simulink model "ellipsoidSMC"  (R2024a)
settings: Solver=ode45  StartTime=0  StopTime=350  FixedStep=0.01  MaxStep=0.01  RelTol=1e-4  AbsTol=1e-4  EnableMultiTasking=on
values from neighbouring files (symbols this model uses):
  simu = simulationClass()    [wecSimInputFile.m]
  waves = waveClass('regular')    [wecSimInputFile.m]
undefined symbols (not defined in the file or in its folder): body, controller, pto, X, Y, Z
libraries: nesl_utility x22, sm_lib x16, WECSim_Lib_Body_Elements x6, WECSim_Lib_Frames x1, vrlib x1, WECSim_Lib_PTOs x1
(part 3 of 3)

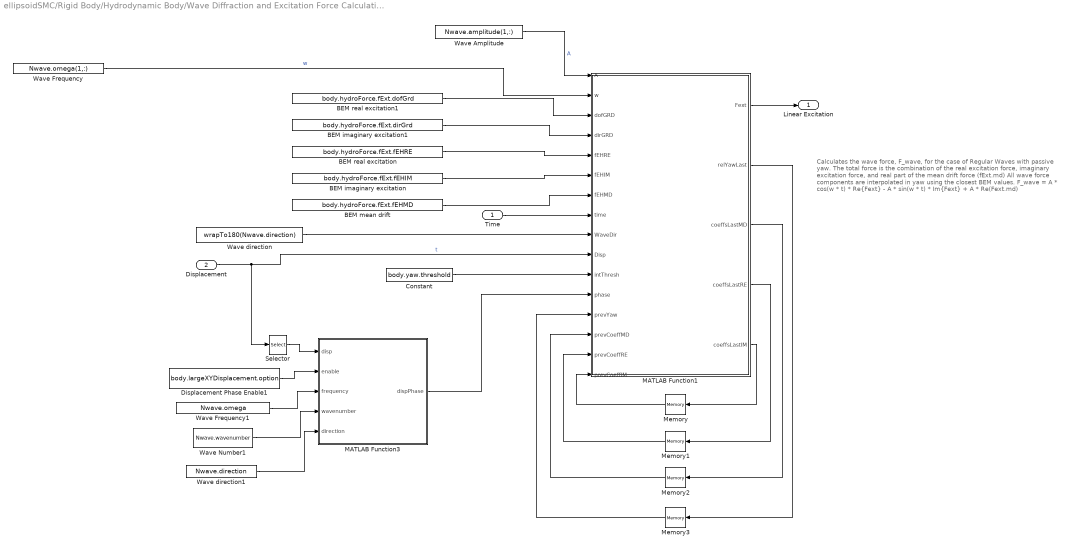
== system ellipsoidSMC/Rigid Body/Hydrodynamic Body/Wave Diffraction and Excitation Force Calculation/Linear Wave Excitation Force Variant Subsystem/Regular Wave NonLinear Yaw ==
  note: Calculates the wave force, F_wave, for the case of Regular Waves with passive yaw.
      |
      | The total force is the combination of the real excitation force, imaginary excitation force, and real part of the mean drift force (fExt.md)
      |
      | All wave force components are interpolated in yaw using the closest BEM values.
      |
      | F_wave =   A * cos(w * t) * Re{Fext}
      |                -  A * sin(w * t) * Im{Fext}
      |                + A * Re(Fext.md)
  Time : Inport
  Displacement : Inport  Port=2
  BEM imaginary excitation : Constant  Value=body.hydroForce.fExt.fEHIM  VectorParams1D=off
  BEM imaginary excitation1 : Constant  Value=body.hydroForce.fExt.dirGrd  VectorParams1D=off
  BEM mean drift : Constant  Value=body.hydroForce.fExt.fEHMD  VectorParams1D=off
  BEM real excitation : Constant  Value=body.hydroForce.fExt.fEHRE  VectorParams1D=off
  BEM real excitation1 : Constant  Value=body.hydroForce.fExt.dofGrd  VectorParams1D=off
  Constant : Constant  Value=body.yaw.threshold
  Displacement Phase Enable1 : Constant  Value=body.largeXYDisplacement.option
  MATLAB Function1 : MATLAB Function  TreatAsAtomicUnit=on
  MATLAB Function3 : MATLAB Function  TreatAsAtomicUnit=on
  Memory{,1..3} (4 alike) : Memory  InheritSampleTime=on  LinearizeAsDelay=on
  Selector : Selector  IndexOptions=Index vector (dialog)  Indices=[1 2]  OutputSizes=1
  Wave Amplitude : Constant  Value=Nwave.amplitude(1,:)
  Wave Frequency : Constant  Value=Nwave.omega(1,:)
  Wave Frequency1 : Constant  Value=Nwave.omega  VectorParams1D=off
  Wave Number1 : Constant  Value=Nwave.wavenumber
  Wave direction : Constant  Value=wrapTo180(Nwave.direction)  VectorParams1D=off
  Wave direction1 : Constant  Value=Nwave.direction  VectorParams1D=off
  Linear Excitation : Outport
  wires:
  Wave Frequency1/1 -> MATLAB Function3/3(frequency)
  Selector/1 -> MATLAB Function3/1(disp)
  Displacement Phase Enable1/1 -> MATLAB Function3/2(enable)
  Wave Number1/1 -> MATLAB Function3/4(wavenumber)
  Displacement/1 -> Selector/1, MATLAB Function1/10(Disp)  "t"
  Wave direction1/1 -> MATLAB Function3/5(direction)
  MATLAB Function3/1(dispPhase) -> MATLAB Function1/12(phase)
  Time/1 -> MATLAB Function1/8(time)
  MATLAB Function1/1(Fext) -> Linear Excitation/1
  Wave Frequency/1 -> MATLAB Function1/2(w)  "w"
  MATLAB Function1/5(coeffsLastIM) -> Memory/1
  MATLAB Function1/2(relYawLast) -> Memory3/1
  MATLAB Function1/4(coeffsLastRE) -> Memory1/1
  Memory3/1 -> MATLAB Function1/13(prevYaw)
  BEM mean drift/1 -> MATLAB Function1/7(fEHMD)
  Memory/1 -> MATLAB Function1/16(prevCoeffIM)
  Wave Amplitude/1 -> MATLAB Function1/1(A)  "A"
  MATLAB Function1/3(coeffsLastMD) -> Memory2/1
  BEM real excitation/1 -> MATLAB Function1/5(fEHRE)
  Wave direction/1 -> MATLAB Function1/9(WaveDir)
  BEM imaginary excitation/1 -> MATLAB Function1/6(fEHIM)
  BEM real excitation1/1 -> MATLAB Function1/3(dofGRD)
  Memory1/1 -> MATLAB Function1/15(prevCoeffRE)
  BEM imaginary excitation1/1 -> MATLAB Function1/4(dirGRD)
  Constant/1 -> MATLAB Function1/11(intThresh)
  Memory2/1 -> MATLAB Function1/14(prevCoeffMD)

== system ellipsoidSMC/Rigid Body/Hydrodynamic Body/Wave Diffraction and Excitation Force Calculation/Linear Wave Excitation Force Variant Subsystem/User Defined Wave Excitation Force ==
  note: Calculates the wave force, F_wave, for the case of User Defined Waves.
      |
      | F_wave = convolution calculation [1x6]
  InputWaveForceTimeHistory : FromWorkspace  VariableName=[Nwave.waveAmpTime(:,1),body.hydroForce.userDefinedFe]
  Linear Excitation : Outport
  wires:
  InputWaveForceTimeHistory/1 -> Linear Excitation/1

== system ellipsoidSMC/Rigid Body/Hydrodynamic Body/Wave Diffraction and Excitation Force Calculation/Nonlinear FK Force Variant Subsystem/No Nonlinear FroudeKrylov Force ==
  Constant : Constant  Value=zeros(1,body.dof)
  Nonlinear Excitation : Outport
  wires:
  Constant/1 -> Nonlinear Excitation/1

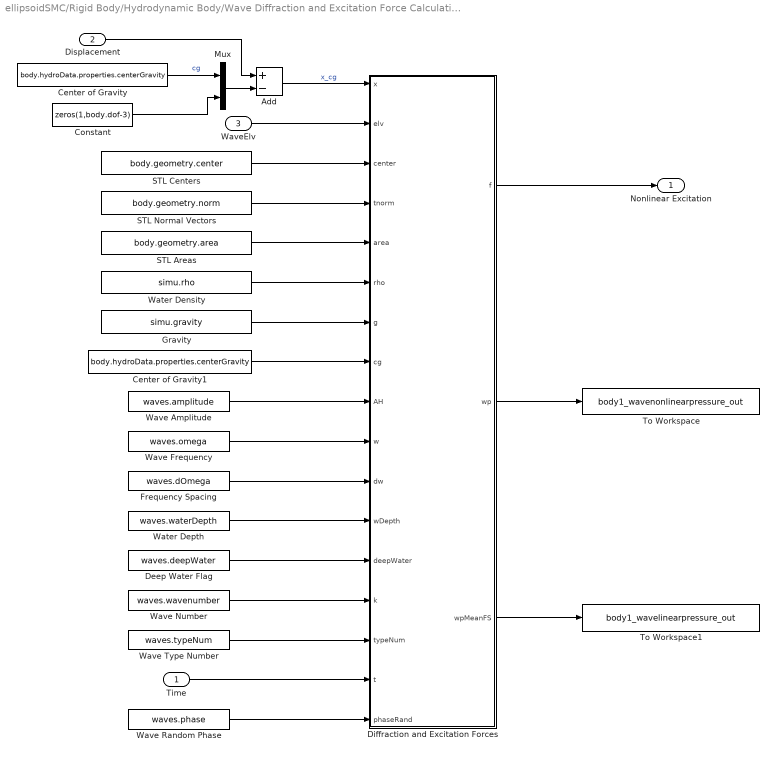
== system ellipsoidSMC/Rigid Body/Hydrodynamic Body/Wave Diffraction and Excitation Force Calculation/Nonlinear FK Force Variant Subsystem/With Nonlinear FroudeKrylov Force ==
  Time : Inport
  Displacement : Inport  Port=2
  WaveElv : Inport  Port=3
  Add : Sum  Inputs=+-
  Center of Gravity : Constant  Value=body.hydroData.properties.centerGravity
  Center of Gravity1 : Constant  Value=body.hydroData.properties.centerGravity
  Constant : Constant  Value=zeros(1,body.dof-3)
  Deep Water Flag : Constant  Value=waves.deepWater
  Diffraction and Excitation Forces : MATLAB Function  TreatAsAtomicUnit=on
  Frequency Spacing : Constant  Value=waves.dOmega
  Gravity : Constant  Value=simu.gravity
  Mux : Mux  Inputs=2
  STL Areas : Constant  Value=body.geometry.area
  STL Centers : Constant  Value=body.geometry.center
  STL Normal Vectors : Constant  Value=body.geometry.norm
  To Workspace : ToWorkspace  VariableName=body1_wavenonlinearpressure_out  SaveFormat=Structure With Time  SampleTime=-1
      settings: Decimation=round(simu.dtOut/simu.dt,0)
  To Workspace1 : ToWorkspace  VariableName=body1_wavelinearpressure_out  SaveFormat=Structure With Time  SampleTime=-1
      settings: Decimation=round(simu.dtOut/simu.dt,0)
  Water Density : Constant  Value=simu.rho
  Water Depth : Constant  Value=waves.waterDepth
  Wave Amplitude : Constant  Value=waves.amplitude
  Wave Frequency : Constant  Value=waves.omega
  Wave Number : Constant  Value=waves.wavenumber
  Wave Random Phase : Constant  Value=waves.phase
  Wave Type Number : Constant  Value=waves.typeNum
  Nonlinear Excitation : Outport
  wires:
  STL Areas/1 -> Diffraction and Excitation Forces/5(area)
  Diffraction and Excitation Forces/2(wp) -> To Workspace/1
  Diffraction and Excitation Forces/3(wpMeanFS) -> To Workspace1/1
  Displacement/1 -> Add/1
  Constant/1 -> Mux/2
  Center of Gravity/1 -> Mux/1  "cg"
  Mux/1 -> Add/2
  Add/1 -> Diffraction and Excitation Forces/1(x)  "x_cg"
  Deep Water Flag/1 -> Diffraction and Excitation Forces/13(deepWater)
  Wave Random Phase/1 -> Diffraction and Excitation Forces/17(phaseRand)
  Water Depth/1 -> Diffraction and Excitation Forces/12(wDepth)
  Wave Number/1 -> Diffraction and Excitation Forces/14(k)
  Wave Type Number/1 -> Diffraction and Excitation Forces/15(typeNum)
  Frequency Spacing/1 -> Diffraction and Excitation Forces/11(dw)
  Wave Frequency/1 -> Diffraction and Excitation Forces/10(w)
  Wave Amplitude/1 -> Diffraction and Excitation Forces/9(AH)
  Time/1 -> Diffraction and Excitation Forces/16(t)
  WaveElv/1 -> Diffraction and Excitation Forces/2(elv)
  STL Centers/1 -> Diffraction and Excitation Forces/3(center)
  STL Normal Vectors/1 -> Diffraction and Excitation Forces/4(tnorm)
  Water Density/1 -> Diffraction and Excitation Forces/6(rho)
  Gravity/1 -> Diffraction and Excitation Forces/7(g)
  Diffraction and Excitation Forces/1(f) -> Nonlinear Excitation/1
  Center of Gravity1/1 -> Diffraction and Excitation Forces/8(cg)

== system ellipsoidSMC/Rigid Body/Hydrodynamic Body/Wave Radiation Forces Calculation/SS CI and Constant-Damping-CoeVariant Subsystem/Constant Coefficients ==
  note: F = damping * velocity
  velocity : Inport
  Product : Product  Multiplication=Matrix(*)
  Radiation Damping Matrix : Constant  Value=body.hydroForce.fDamping
  Out1 : Outport
  wires:
  velocity/1 -> Product/2
  Product/1 -> Out1/1  "F_Single Frequency"
  Radiation Damping Matrix/1 -> Product/1

== system ellipsoidSMC/Rigid Body/Hydrodynamic Body/Wave Radiation Forces Calculation/SS CI and Constant-Damping-CoeVariant Subsystem/Convolution Integral Calculation ==
  note: Calculate the convolution integral using the radiation IRF (body.hydroForce.irkb) and the velocity.
  velocity : Inport
  IRBK : Constant  Value=body.hydroForce.irkb
  MATLAB Function1 : MATLAB Function  TreatAsAtomicUnit=on  SystemSampleTime=simu.cicTime(2)-simu.cicTime(1)
  Rate Transition : RateTransition
  Reshape : Reshape
  cicTime : Constant  Value=simu.cicTime
  Out1 : Outport
  wires:
  velocity/1 -> MATLAB Function1/1(velocity)
  cicTime/1 -> MATLAB Function1/3(cicTime)
  IRBK/1 -> MATLAB Function1/2(IRKB)
  MATLAB Function1/1(F_FM) -> Rate Transition/1
  Rate Transition/1 -> Reshape/1
  Reshape/1 -> Out1/1

== system ellipsoidSMC/Rigid Body/Hydrodynamic Body/Wave Radiation Forces Calculation/SS CI and Constant-Damping-CoeVariant Subsystem/FIR Filter Calculation ==
  velocity : Inport
  FIR Filter Matrix : Subsystem  mask{B2B=simu.b2b, body=body}
      mask prompts: body "bodyClass"
      mask init:
      | if exist('body','var')
      |     TotalRows = body.dof;
      |     
      |     cb = gcb;
      |     
      |     set_param([cb '/Mux'],...
      |                'Inputs',sprintf('%d',TotalRows));
      |     
      |     set_param([cb '/FIR_filter_row'],...
      |                'position',[0, 100, 200, 140]);
      |     
      |     set_param([cb '/FIR_filter_row'],...
      |                'rowNo', '1');
      |     
      |     try
      |     add_line(cb,...
      |             ['velocity','/1'], ...    
      |             'FIR_filter_row/1',... 
      |             'autorouting','on');
      |     catch
      |     end
      |     
      |     try
      |     add_line(cb,...
      |             ['FIR_filter_row','/1'], ...    
      |             'Mux/1',... 
      |             'autorouting','on');
      |     catch
      |     end
      |     
      |     for i = 2:TotalRows
      |         add_block([cb,'/FIR_filter_row'],[cb,'/FIR_filter_row',num2str(i)], 'MakeNameUnique','off');
      |         set_param([cb '/FIR_filter_row',num2str(i)],...
      |                    'position',[0, 100*i, 200, 40 + 100*i]);
      |         set_param([cb '/FIR_filter_row',num2str(i)],...
      |                    'rowNo', num2str(i));
      |         add_line(cb,...
      |                 ['velocity','/1'], ...    
      |                 ['FIR_filter_row',num2str(i),'/1'],... 
      |                 'autorouting','on');
      |         add_line(cb,...
      |                 ['FIR_filter_row',num2str(i),'/1'], ...    
      |                 ['Mux/',num2str(i)],... 
      |                 'autorouting','on');
      |     end
      | end
  Rate Transition : RateTransition  OutPortSampleTime=simu.cicDt
  Rate Transition1 : RateTransition  OutPortSampleTime=simu.cicDt
  Out1 : Outport
  wires:
  Rate Transition1/1 -> Out1/1
  Rate Transition/1 -> FIR Filter Matrix/1(velocity)
  FIR Filter Matrix/1(Out1) -> Rate Transition1/1
  velocity/1 -> Rate Transition/1

== system ellipsoidSMC/Rigid Body/Hydrodynamic Body/Wave Radiation Forces Calculation/SS CI and Constant-Damping-CoeVariant Subsystem/State-Space Calculation  ==
  note: Calculate the radiation damping based on the state space formulation. Coefficients are defined in body.hydroForce.ssRadf
  velocity : Inport
  State-Space : StateSpace  A=body.hydroForce.ssRadf.A  B=body.hydroForce.ssRadf.B  C=body.hydroForce.ssRadf.C  D=body.hydroForce.ssRadf.D  InitialCondition=0
  Out1 : Outport
  wires:
  State-Space/1 -> Out1/1
  velocity/1 -> State-Space/1  "x"

== system ellipsoidSMC/Rigid Body/Hydrodynamic Body/Hydrostatic Restoring Force Calculation/Linear and Nonlinear Restoring Force Variant Subsystem/Linear Hydrostatic Restoring Force/Net Buoyancy Force ==
  note: The total buoyancy force is due to the vertical buoyancy force (gravity - buoyancy) and a rotational buoyancy force if the center of gravity is not aligned with the center of buoyancy.
      |
      | F_NetBuoyancy = F_gravity - F_buoyancy + F_rotational_buoyancy
      |
      | F_rotational_buoyancy = (cb-cg) x F_buoyancy
      | F_buoyancy = rho*g*V_0
      | F_gravity = m*g
  Body Mass : Inport
  Add1 : Sum  Inputs=+-
  Add2 : Sum
  Add3 : Sum  Inputs=+-
  Assignment (Add Net Bouyancy Force to Z-Direction) : Assignment  IndexOptions=Index vector (dialog)  Indices=3  OutputSizes=1
  Assignment (Add Net Bouyancy Force to Z-Direction)1 : Assignment  IndexOptions=Index vector (dialog)  Indices=3  OutputSizes=1
  Assignment (Add Net Bouyancy Force to Z-Direction)2 : Assignment  IndexOptions=Index vector (dialog)  Indices=4:6  OutputSizes=1
  Center of Buoyancy : Constant  Value=body.centerBuoyancy
  Center of Gravity : Constant  Value=body.centerGravity
  Constant1 : Constant  Value=zeros(1,body.dof)
  Constant2 : Constant  Value=[0 0 0]
  Cross Product : vrlib/Utilities/Cross Product
  Gravity : Constant  Value=simu.gravity
  Product : Product
  Product1 : Product  Inputs=3
  Volume : Constant  Value=body.volume
  Water Density : Constant  Value=simu.rho
  F_NetBuoyancy : Outport
  wires:
  Add1/1 -> Assignment (Add Net Bouyancy Force to Z-Direction)/2
  Body Mass/1 -> Product/2  "m"
  Cross Product/1 -> Assignment (Add Net Bouyancy Force to Z-Direction)2/2
  Add2/1 -> F_NetBuoyancy/1  "Net buoyancy force"
  Add3/1 -> Cross Product/2
  Constant2/1 -> Assignment (Add Net Bouyancy Force to Z-Direction)1/1
  Center of Gravity/1 -> Add3/2  "cg"
  Constant1/1 -> Assignment (Add Net Bouyancy Force to Z-Direction)/1, Assignment (Add Net Bouyancy Force to Z-Direction)2/1
  Center of Buoyancy/1 -> Add3/1  "x"
  Assignment (Add Net Bouyancy Force to Z-Direction)1/1 -> Cross Product/1
  Volume/1 -> Product1/3  "Vol"
  Assignment (Add Net Bouyancy Force to Z-Direction)/1 -> Add2/1  "Vertical Buoyancy Force"
  Water Density/1 -> Product1/1  "rho"
  Gravity/1 -> Product/1, Product1/2  "g"
  Product1/1 -> Assignment (Add Net Bouyancy Force to Z-Direction)1/2, Add1/2  "F_Buoyancy"
  Product/1 -> Add1/1  "F_Gravity"
  Assignment (Add Net Bouyancy Force to Z-Direction)2/1 -> Add2/2  "Rotational buoyancy force"

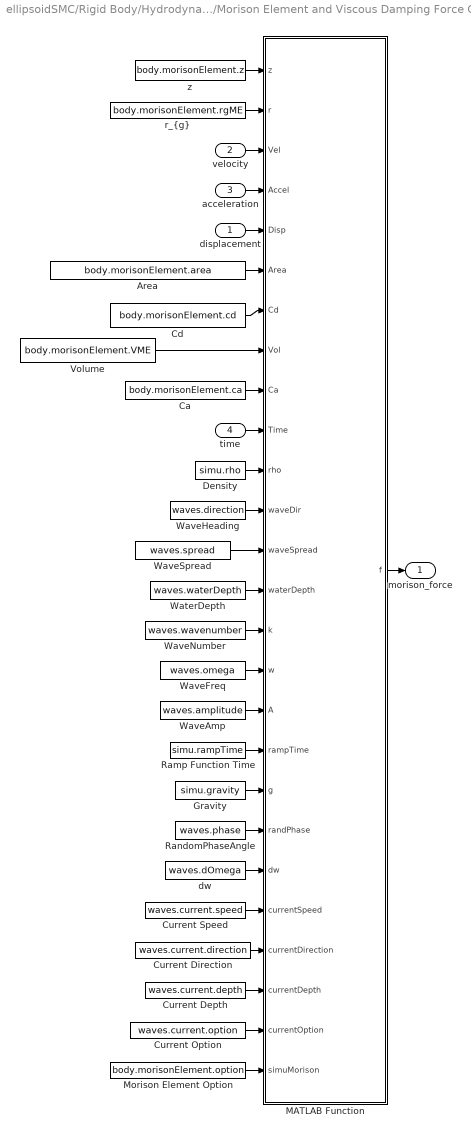
== system ellipsoidSMC/Rigid Body/Hydrodynamic Body/Morison Element and Viscous Damping Force Calculation/Morison Element Variant Subsystem/Morison Element On/Irregular Wave Morison Force ==
  displacement : Inport
  velocity : Inport  Port=2
  acceleration : Inport  Port=3
  time : Inport  Port=4
  Area : Constant  Value=body.morisonElement.area  VectorParams1D=off
  Ca : Constant  Value=body.morisonElement.ca  VectorParams1D=off
  Cd : Constant  Value=body.morisonElement.cd  VectorParams1D=off
  Current Depth : Constant  Value=waves.current.depth
  Current Direction : Constant  Value=waves.current.direction
  Current Option : Constant  Value=waves.current.option
  Current Speed : Constant  Value=waves.current.speed
  Density : Constant  Value=simu.rho
  Gravity : Constant  Value=simu.gravity
  MATLAB Function : MATLAB Function  TreatAsAtomicUnit=on
  Morison Element Option : Constant  Value=body.morisonElement.option
  Ramp Function Time : Constant  Value=simu.rampTime
  RandomPhaseAngle : Constant  Value=waves.phase  VectorParams1D=off
  Volume : Constant  Value=body.morisonElement.VME  VectorParams1D=off
  WaterDepth : Constant  Value=waves.waterDepth
  WaveAmp : Constant  Value=waves.amplitude
  WaveFreq : Constant  Value=waves.omega
  WaveHeading : Constant  Value=waves.direction
  WaveNumber : Constant  Value=waves.wavenumber
  WaveSpread : Constant  Value=waves.spread
  dw : Constant  Value=waves.dOmega  VectorParams1D=off
  "r_{g}" : Constant  Value=body.morisonElement.rgME  VectorParams1D=off
  z : Constant  Value=body.morisonElement.z  VectorParams1D=off
  morison_force : Outport
  wires:
  WaveSpread/1 -> MATLAB Function/13(waveSpread)
  Morison Element Option/1 -> MATLAB Function/26(simuMorison)
  Current Option/1 -> MATLAB Function/25(currentOption)
  Current Depth/1 -> MATLAB Function/24(currentDepth)
  Current Direction/1 -> MATLAB Function/23(currentDirection)
  Current Speed/1 -> MATLAB Function/22(currentSpeed)
  dw/1 -> MATLAB Function/21(dw)
  RandomPhaseAngle/1 -> MATLAB Function/20(randPhase)
  Gravity/1 -> MATLAB Function/19(g)
  Ramp Function Time/1 -> MATLAB Function/18(rampTime)
  WaveAmp/1 -> MATLAB Function/17(A)
  WaveFreq/1 -> MATLAB Function/16(w)
  WaveNumber/1 -> MATLAB Function/15(k)
  WaterDepth/1 -> MATLAB Function/14(waterDepth)
  WaveHeading/1 -> MATLAB Function/12(waveDir)
  Density/1 -> MATLAB Function/11(rho)
  time/1 -> MATLAB Function/10(Time)
  Ca/1 -> MATLAB Function/9(Ca)
  Volume/1 -> MATLAB Function/8(Vol)
  Cd/1 -> MATLAB Function/7(Cd)
  Area/1 -> MATLAB Function/6(Area)
  displacement/1 -> MATLAB Function/5(Disp)
  acceleration/1 -> MATLAB Function/4(Accel)
  velocity/1 -> MATLAB Function/3(Vel)
  "r_{g}"/1 -> MATLAB Function/2(r)
  z/1 -> MATLAB Function/1(z)
  MATLAB Function/1(f) -> morison_force/1

== system ellipsoidSMC/Rigid Body/Hydrodynamic Body/Morison Element and Viscous Damping Force Calculation/Morison Element Variant Subsystem/Morison Element On/No Wave Morison Force ==
  displacement : Inport
  velocity : Inport  Port=2
  acceleration : Inport  Port=3
  time : Inport  Port=4
  Area : Constant  Value=body.morisonElement.area  VectorParams1D=off
  Ca : Constant  Value=body.morisonElement.ca  VectorParams1D=off
  Cd : Constant  Value=body.morisonElement.cd  VectorParams1D=off
  Current Depth : Constant  Value=waves.current.depth
  Current Direction : Constant  Value=waves.current.direction
  Current Option : Constant  Value=waves.current.option
  Current Speed : Constant  Value=waves.current.speed
  Density : Constant  Value=simu.rho
  Morison Element Option : Constant  Value=body.morisonElement.option
  MorisonElement(s) : MATLAB Function  TreatAsAtomicUnit=on
  Ramp Function Time : Constant  Value=simu.rampTime
  Volume : Constant  Value=body.morisonElement.VME  VectorParams1D=off
  "r_{g}" : Constant  Value=body.morisonElement.rgME  VectorParams1D=off
  z : Constant  Value=body.morisonElement.z  VectorParams1D=off
  morison_force : Outport
  wires:
  Morison Element Option/1 -> MorisonElement(s)/17(bodyMorison)
  Current Option/1 -> MorisonElement(s)/16(currentOption)
  Current Depth/1 -> MorisonElement(s)/15(currentDepth)
  Current Direction/1 -> MorisonElement(s)/14(currentDirection)
  Current Speed/1 -> MorisonElement(s)/13(currentSpeed)
  Ramp Function Time/1 -> MorisonElement(s)/12(rampTime)
  Density/1 -> MorisonElement(s)/11(rho)
  time/1 -> MorisonElement(s)/10(Time)
  Ca/1 -> MorisonElement(s)/9(Ca)
  Volume/1 -> MorisonElement(s)/8(Vol)
  Cd/1 -> MorisonElement(s)/7(Cd)
  Area/1 -> MorisonElement(s)/6(Area)
  displacement/1 -> MorisonElement(s)/5(Disp)
  acceleration/1 -> MorisonElement(s)/4(Accel)
  velocity/1 -> MorisonElement(s)/3(Vel)
  "r_{g}"/1 -> MorisonElement(s)/2(r)
  z/1 -> MorisonElement(s)/1(z)
  MorisonElement(s)/1(f) -> morison_force/1

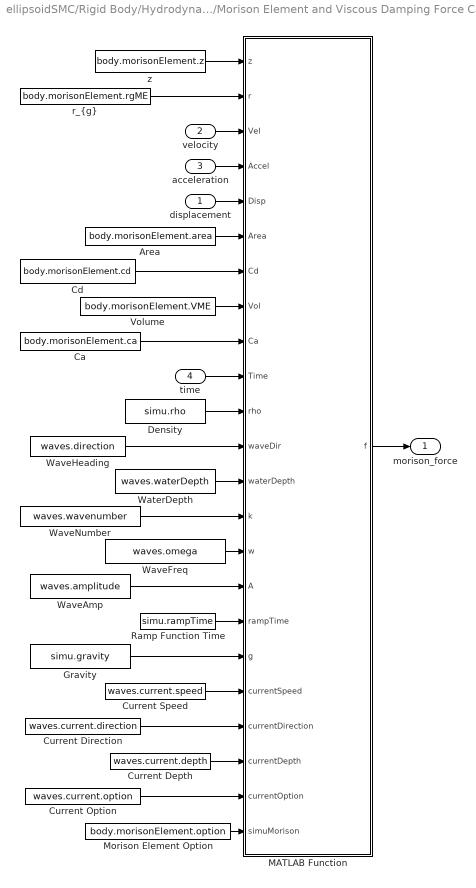
== system ellipsoidSMC/Rigid Body/Hydrodynamic Body/Morison Element and Viscous Damping Force Calculation/Morison Element Variant Subsystem/Morison Element On/Regular Wave Morison Force ==
  displacement : Inport
  velocity : Inport  Port=2
  acceleration : Inport  Port=3
  time : Inport  Port=4
  Area : Constant  Value=body.morisonElement.area  VectorParams1D=off
  Ca : Constant  Value=body.morisonElement.ca  VectorParams1D=off
  Cd : Constant  Value=body.morisonElement.cd  VectorParams1D=off
  Current Depth : Constant  Value=waves.current.depth
  Current Direction : Constant  Value=waves.current.direction
  Current Option : Constant  Value=waves.current.option
  Current Speed : Constant  Value=waves.current.speed
  Density : Constant  Value=simu.rho
  Gravity : Constant  Value=simu.gravity
  MATLAB Function : MATLAB Function  TreatAsAtomicUnit=on
  Morison Element Option : Constant  Value=body.morisonElement.option
  Ramp Function Time : Constant  Value=simu.rampTime
  Volume : Constant  Value=body.morisonElement.VME  VectorParams1D=off
  WaterDepth : Constant  Value=waves.waterDepth
  WaveAmp : Constant  Value=waves.amplitude
  WaveFreq : Constant  Value=waves.omega
  WaveHeading : Constant  Value=waves.direction
  WaveNumber : Constant  Value=waves.wavenumber
  "r_{g}" : Constant  Value=body.morisonElement.rgME  VectorParams1D=off
  z : Constant  Value=body.morisonElement.z  VectorParams1D=off
  morison_force : Outport
  wires:
  Current Speed/1 -> MATLAB Function/19(currentSpeed)
  WaveAmp/1 -> MATLAB Function/16(A)
  Gravity/1 -> MATLAB Function/18(g)
  WaveNumber/1 -> MATLAB Function/14(k)
  Ca/1 -> MATLAB Function/9(Ca)
  Current Direction/1 -> MATLAB Function/20(currentDirection)
  Area/1 -> MATLAB Function/6(Area)
  WaterDepth/1 -> MATLAB Function/13(waterDepth)
  acceleration/1 -> MATLAB Function/4(Accel)
  Density/1 -> MATLAB Function/11(rho)
  WaveHeading/1 -> MATLAB Function/12(waveDir)
  WaveFreq/1 -> MATLAB Function/15(w)
  Cd/1 -> MATLAB Function/7(Cd)
  displacement/1 -> MATLAB Function/5(Disp)
  Current Option/1 -> MATLAB Function/22(currentOption)
  Current Depth/1 -> MATLAB Function/21(currentDepth)
  time/1 -> MATLAB Function/10(Time)
  "r_{g}"/1 -> MATLAB Function/2(r)
  Ramp Function Time/1 -> MATLAB Function/17(rampTime)
  velocity/1 -> MATLAB Function/3(Vel)
  Volume/1 -> MATLAB Function/8(Vol)
  Morison Element Option/1 -> MATLAB Function/23(simuMorison)
  z/1 -> MATLAB Function/1(z)
  MATLAB Function/1(f) -> morison_force/1

== system ellipsoidSMC/Rigid Body/Hydrodynamic Body/Wave Radiation Forces Calculation/SS CI and Constant-Damping-CoeVariant Subsystem/FIR Filter Calculation/FIR Filter Matrix ==
  velocity : Inport
  FIR_filter_row : Subsystem  mask{body=body, B2B=simu.b2b, rowNo=1}
      mask prompts: body "BodyClass"
      mask init:
      | cb = gcb;
      | % The implementation that follows, calculates the radiation force, Fr, by
      | % calculating the Fr for each body mode by multiplying the velocity vector
      | % to the IRF matrix -- whose each row corresponds to the Fr for each of the
      | % modes corresponding to the velocity vector.
      | 
      | 
      | % Get the radiation IRF coefficients using body.hydroForce.irkb
      | set_param([cb '/Discrete FIR Filter'],...
      |            'position',[100, 0, 140, 180]);
      |          if rem(rowNo,6) ~= 0
      |         set_param([cb,'/Discrete FIR Filter'],...
      |                   'Coefficients', [sprintf('transpose(squeeze(body.hydroForce.irkb(:,%d,%d)))',rem(rowNo,6),1)]); 
      |          elseif rem(rowNo,6) == 0
      |         set_param([cb,'/Discrete FIR Filter'],...
      |                   'Coefficients', [sprintf('transpose(squeeze(body.hydroForce.irkb(:,%d,%d)))',6,1)]); 
      |          end
      | % Assign number of filters. The number of filter corresponds to the IRF
      | % matrix elements being used for the calculation for each row.
      | nFilt = body.dof + B2B*(body.total-1)*6;
      | 
      | % Add Demux channels corresponding to number of filters, and connect them to the corresponding filter.
      | 
      | set_param([cb '/Demux'],...
      |            'Outputs',sprintf('%d',nFilt));
      | try
      | add_line(cb,...
      |         'Demux/1',...
      |         ['Discrete FIR Filter','/1'], ...     
      |         'autorouting','on');
      | catch
      | end
      | 
      | try
      | add_line(cb,...
      |         'Discrete FIR Filter/1', ...     
      |         'Add/1',...
      |         'autorouting','on');
      | catch 
      | end
      | 
      | % Add filters 
      | 
      | for i = 2:nFilt
      | 
      |      try
      |         add_block([cb,'/Discrete FIR Filter'],[cb,'/Discrete FIR Filter ',num2str(i)],'MakeNameUnique','off',...
      |                    'Position',[100*i, 0, 40+100*i, 180],'BackgroundColor','white');
      |         signlist = get_param([cb,'/Add'],'Inputs');
      |         set_param([cb,'/Add'],'Inputs',[signlist,'+']);
      |      catch 
      |      end
      | 
      | 
      |      try
      |          if rem(rowNo,6) ~= 0
      |         set_param([cb,'/Discrete FIR Filter ',num2str(i)],...
      |                   'Coefficients', [sprintf('transpose(squeeze(body.hydroForce.irkb(:,%d,%d)))',rem(rowNo,6),i)]); 
      |          elseif rem(rowNo,6) == 0
      |         set_param([cb,'/Discrete FIR Filter ',num2str(i)],...
      |                   'Coefficients', [sprintf('transpose(squeeze(body.hydroForce.irkb(:,%d,%d)))',6,i)]); 
      |          end
      |      catch
      |      end
      | 
      |      try
      |         add_line(cb,...
      |         ['Demux/',num2str(i)],...
      |         ['Discrete FIR Filter ',num2str(i),'/1'], ...     
      |         'autorouting','on');
      |      catch
      |      end
      | 
      | 
      |      try
      |         add_line(cb,...
      |         ['Discrete FIR Filter ',num2str(i),'/1'], ...     
      |         ['Add/', num2str(i)],...
      |         'autorouting','on');
      |     catch 
      |     end
      | end
  Gain : Gain  Gain=simu.cicDt
  Mux : Mux  Inputs=1
  Out1 : Outport
  wires:
  Gain/1 -> Out1/1
  FIR_filter_row/1(Out1) -> Mux/1
  velocity/1 -> FIR_filter_row/1(In1)
  Mux/1 -> Gain/1

== system ellipsoidSMC/Rigid Body/Hydrodynamic Body/Wave Radiation Forces Calculation/SS CI and Constant-Damping-CoeVariant Subsystem/FIR Filter Calculation/FIR Filter Matrix/FIR_filter_row ==
  In1 : Inport
  Add : Sum  Inputs=+
  Demux : Demux  Outputs=1
      settings: AttributesFormatString=%<Outputs>
  Discrete FIR Filter : DiscreteFir  Coefficients=transpose(squeeze(body.hydroForce.irkb(:,1,1)))
  Out1 : Outport
  wires:
  Add/1 -> Out1/1
  In1/1 -> Demux/1

== matlab function ellipsoidSMC/Rigid Body/Hydrodynamic Body/Morison Element and Viscous Damping Force Calculation/Morison Element Variant Subsystem/Morison Element On/No Wave Morison Force/MorisonElement(s) ==
  data: z input; f output; r input; Vel input; Accel input; Disp input; Area input; Cd input; Vol input; Ca input; Time input; rho input; rampTime input; currentSpeed input; currentDirection input; currentDepth input; currentOption input; bodyMorison input
function f = noWaveMorison(z,r,Vel,Accel,Disp,Area,Cd,Vol,Ca,Time,rho,rampTime,currentSpeed,currentDirection,currentDepth,currentOption,bodyMorison)

f = noWaveMorison(z,r,Vel,Accel,Disp,Area,Cd,Vol,Ca,Time,rho,rampTime,currentSpeed,currentDirection,currentDepth,currentOption,bodyMorison);

end

== matlab function ellipsoidSMC/Rigid Body/Hydrodynamic Body/Morison Element and Viscous Damping Force Calculation/Morison Element Variant Subsystem/Morison Element On/Irregular Wave Morison Force/MATLAB Function ==
  data: z input; f output; r input; Vel input; Accel input; Disp input; Area input; Cd input; Vol input; Ca input; Time input; rho input; waveDir input; waveSpread input; waterDepth input; k input; w input; A input; rampTime input; g input; randPhase input; dw input; currentSpeed input; currentDirection input; currentDepth input; currentOption input; simuMorison input
function f = irregWaveMorison(z,r,Vel,Accel,Disp,Area,Cd,Vol,Ca,Time,rho,waveDir,waveSpread,waterDepth,k,w,A,rampTime,g,randPhase,dw,currentSpeed,currentDirection,currentDepth,currentOption,simuMorison)

f = irregWaveMorison(z,r,Vel,Accel,Disp,Area,Cd,Vol,Ca,Time,rho,waveDir,waveSpread,waterDepth,k,w,A,rampTime,g,randPhase,dw,currentSpeed,currentDirection,currentDepth,currentOption,simuMorison);

end

== matlab function ellipsoidSMC/Rigid Body/Hydrodynamic Body/Wave Diffraction and Excitation Force Calculation/Linear Wave Excitation Force Variant Subsystem/Irregular Wave Excitation Force/MATLAB Function2 ==
  data: disp input; dispPhase output; enable input; frequency input; wavenumber input; direction input
function dispPhase  = calcDispPhase(disp, enable, frequency, wavenumber, direction)
% initialize
dispPhase = zeros(length(frequency),length(direction));
% execute
dispPhase = calcDispPhase(disp, enable, direction, frequency, wavenumber);

end

== matlab function ellipsoidSMC/Rigid Body/Hydrodynamic Body/Wave Diffraction and Excitation Force Calculation/Linear Wave Excitation Force Variant Subsystem/Regular Wave NonLinear Yaw/MATLAB Function3 ==
  data: disp input; dispPhase output; enable input; frequency input; wavenumber input; direction input
function dispPhase  = calcDispPhase(disp, enable, frequency, wavenumber, direction)
% initialize
dispPhase = zeros(length(frequency),length(direction));
% execute
dispPhase = calcDispPhase(disp, enable, direction, frequency, wavenumber);

end

== matlab function ellipsoidSMC/Rigid Body/Hydrodynamic Body/Wave Diffraction and Excitation Force Calculation/Linear Wave Excitation Force Variant Subsystem/Regular Wave Excitation Force/MATLAB Function1 ==
  data: disp input; dispPhase output; enable input; frequency input; wavenumber input; direction input
function dispPhase  = calcDispPhase(disp, enable, frequency, wavenumber, direction)
% initialize
dispPhase = zeros(length(frequency),length(direction));
% execute
dispPhase = calcDispPhase(disp, enable, direction, frequency, wavenumber);

end

== matlab function ellipsoidSMC/Rigid Body/Hydrodynamic Body/Nonlinear Wave Elevation/Linear or Instantaneous Free Surface/Instantaneous Water Free Surface/Instantaneous FS ==
  data: x input; center input; f output; cg input; AH input; w input; dw input; k input; typeNum input; t input; rampT input; phaseRand input; waveDir input
function f  = waveElevation(x,center,cg,AH,w,dw,k,typeNum,t,rampT,phaseRand,waveDir)

f  = waveElevation(x,center,cg,AH,w,dw,k,typeNum,t,rampT,phaseRand,waveDir);

end

== matlab function ellipsoidSMC/Rigid Body/Hydrodynamic Body/Structure/Motion Sensor/quaternion2EulXYZ ==
  data: Q input; E output
function E = quaternion2EulXYZ(Q)

E = quaternion2EulXYZ(Q);

end

== matlab function ellipsoidSMC/Rigid Body/Hydrodynamic Body/Wave Diffraction and Excitation Force Calculation/Linear Wave Excitation Force Variant Subsystem/Irregular Wave Excitation Force/MATLAB Function ==
  data: A input; Fext output; w input; fExtRE input; fExtIM input; phaseRand input; dw input; time input; WaveDir input; spread input; fExtMD input
function Fext = irregExcF(A,w,fExtRE,fExtIM,phaseRand,dw,time,WaveDir,spread,fExtMD)

Fext = irregExcF(A,w,fExtRE,fExtIM,phaseRand,dw,time,WaveDir,spread,fExtMD);

end

== matlab function ellipsoidSMC/Rigid Body/Hydrodynamic Body/Wave Diffraction and Excitation Force Calculation/Nonlinear FK Force Variant Subsystem/With Nonlinear FroudeKrylov Force/Diffraction and Excitation Forces ==
  data: x input; elv input; center input; f output; tnorm input; area input; rho input; g input; cg input; AH input; w input; dw input; wDepth input; deepWater input; k input; typeNum input; t input; phaseRand input; wp output; wpMeanFS output
function [f, wp, wpMeanFS]  = nonFKForce(x,elv,center,tnorm,area,rho,g,cg,AH,w,dw,wDepth,deepWater,k,typeNum,t,phaseRand)

[f, wp, wpMeanFS]  = nonFKForce(x,elv,center,tnorm,area,rho,g,cg,AH,w,dw,wDepth,deepWater,k,typeNum,t,phaseRand);

end

== matlab function ellipsoidSMC/Rigid Body/Hydrodynamic Body/Wave Radiation Forces Calculation/SS CI and Constant-Damping-CoeVariant Subsystem/Convolution Integral Calculation/MATLAB Function1 ==
  data: velocity input; F_FM output; IRKB input; cicTime input
function F_FM = ConvolutionIntegral_interp(velocity, IRKB, cicTime)

F_FM = ConvolutionIntegral_interp(velocity, IRKB, cicTime);

end

== matlab function ellipsoidSMC/Rigid Body/Hydrodynamic Body/Yaw Force Transforms/Yaw Force Transforms ==
  data: yaw input; F_Excitation output; dispGlobal input; F_RadiationDampingLocal input; F_AddedMassLocal input; F_ExcitationLocal input; F_RadiationDamping output; F_RestoringLocal input; F_AddedMass output; F_Restoring output
function [F_Excitation, F_RadiationDamping, F_AddedMass, F_Restoring] = fYawTransforms(yaw, dispGlobal, F_RadiationDampingLocal, F_AddedMassLocal, F_ExcitationLocal, F_RestoringLocal)

[F_Excitation, F_RadiationDamping, F_AddedMass, F_Restoring] = fYawTransforms(yaw, dispGlobal, F_RadiationDampingLocal, F_AddedMassLocal, F_ExcitationLocal, F_RestoringLocal);

end

== matlab function ellipsoidSMC/Rigid Body/Hydrodynamic Body/Wave Diffraction and Excitation Force Calculation/Linear Wave Excitation Force Variant Subsystem/Regular Wave NonLinear Yaw/MATLAB Function1 ==
  data: A input; w input; dofGRD input; dirGRD input; fEHRE input; fEHIM input; Fext output; fEHMD input; time input; WaveDir input; Disp input; intThresh input; phase input; prevYaw input; relYawLast output; prevCoeffMD input; prevCoeffRE input; prevCoeffIM input; coeffsLastMD output; coeffsLastRE output; coeffsLastIM output
function [Fext,relYawLast,coeffsLastMD,coeffsLastRE,coeffsLastIM] = regnLYaw(A,w,dofGRD,dirGRD,fEHRE,fEHIM, fEHMD,time,WaveDir,Disp, intThresh, phase, prevYaw, prevCoeffMD, prevCoeffRE, prevCoeffIM)

%initialize outputs
Fext = zeros(1,6);
relYawLast=0;
coeffsLastMD=zeros(length(w),6); 
coeffsLastRE=zeros(length(w),6);
coeffsLastIM=zeros(length(w),6);

[Fext,relYawLast,coeffsLastMD,coeffsLastRE,coeffsLastIM] = regnLYaw(A,w,dofGRD,dirGRD,fEHRE,fEHIM, fEHMD,time,WaveDir,Disp, intThresh, phase, prevYaw, prevCoeffMD, prevCoeffRE, prevCoeffIM);

end

== matlab function ellipsoidSMC/Rigid Body/Hydrodynamic Body/Yaw Kinematic Transforms/No B2B/Yaw Kinematic Transforms ==
  data: yaw input; dispLoc output; dispGlobal input; velGlobal input; accGlobal input; velLoc output; accLoc output
function [dispLoc, velLoc, accLoc] = kinYawTransform(yaw, dispGlobal, velGlobal, accGlobal)

[dispLoc, velLoc, accLoc] = kinYawTransformNoB2B(yaw, dispGlobal, velGlobal, accGlobal);

end

== matlab function ellipsoidSMC/Rigid Body/Hydrodynamic Body/Yaw Kinematic Transforms/With B2B/Yaw Kinematic Transforms ==
  data: yaw input; dispLoc output; dispGlobal input; velGlobal input; accGlobal input; velLoc output; accLoc output; numBody parameter
function [dispLoc, velLoc, accLoc] = kinYawTransformB2B(yaw, dispGlobal, velGlobal, accGlobal, numBody)

[dispLoc, velLoc, accLoc] = kinYawTransformB2B(yaw, dispGlobal, velGlobal, accGlobal, numBody);

end

== matlab function ellipsoidSMC/Rigid Body/Hydrodynamic Body/Morison Element and Viscous Damping Force Calculation/Morison Element Variant Subsystem/Morison Element On/Regular Wave Morison Force/MATLAB Function ==
  data: z input; f output; r input; Vel input; Accel input; Disp input; Area input; Cd input; Vol input; Ca input; Time input; rho input; waveDir input; waterDepth input; k input; w input; A input; rampTime input; g input; currentSpeed input; currentDirection input; currentDepth input; currentOption input; simuMorison input
function f = regWaveMorison(z,r,Vel,Accel,Disp,Area,Cd,Vol,Ca,Time,rho,waveDir,waterDepth,k,w,A,rampTime,g,currentSpeed,currentDirection,currentDepth,currentOption,simuMorison)

f = regWaveMorison(z,r,Vel,Accel,Disp,Area,Cd,Vol,Ca,Time,rho,waveDir,waterDepth,k,w,A,rampTime,g,currentSpeed,currentDirection,currentDepth,currentOption,simuMorison);

end

== matlab function ellipsoidSMC/Rigid Body/Hydrodynamic Body/Wave Diffraction and Excitation Force Calculation/Linear Wave Excitation Force Variant Subsystem/Irregular Wave NonLinearYaw/MATLAB Function1 ==
  data: disp input; dispPhase output; enable input; frequency input; wavenumber input; direction input
function dispPhase  = calcDispPhase(disp, enable, frequency, wavenumber, direction)
% initialize
dispPhase = zeros(length(frequency),length(direction));
% execute
dispPhase = calcDispPhase(disp, enable, direction, frequency, wavenumber);

end

== matlab function ellipsoidSMC/Rigid Body/Hydrodynamic Body/Hydrostatic Restoring Force Calculation/Linear and Nonlinear Restoring Force Variant Subsystem/Nonlinear Hydrostatic Restoring Force/Restoring Forces ==
  data: x input; elv input; center input; f output; tnorm input; area input; rho input; g input; cg input; p output; mass input
function [f,p]  = nonLinearBuoyancy(x,elv,center,tnorm,area,rho,g,cg,mass)

[f,p]  = nonLinearBuoyancy(x,elv,center,tnorm,area,rho,g,cg,mass);

end

== matlab function ellipsoidSMC/Fuzzy Logic Controller/MATLAB Function ==
  data: Fr input; data1 input; data input; u output; dote input; N44 input; N4 output; a1 input; l input; fi1 input; alfa input; k1 input; k2 input; s output
function [u,N4,s]  = smc_controller(Fr,data1,data,dote,N44,a1,l,fi1,alfa,k1,k2)

% Example usage
Fextc=data;
Fext=data1;
%l=0.001;
m=133918.300000000+199883.890680326;
%a1=83.6;
%fi1=0.8;
%alfa=0.5;
%k1=30;
%k2=20;
s=a1*dote;
%w=0.01; %tan h
%G=(l/a1)*(tanh(w*s));% tanhs replace by sign
%G=(l/a1)*(sign(s));% sign function
%u=(-Fr)+(Fext)-((Fextc)-(G))*(m);% for sign and tanh
%u=(Fr)+(Fext)-(m*Fextc);% for sign and tanh
% %u=(-Fr)+(Fext)+5000000*dote-((Fextc)-(G))*(m);%for 2nd order slidig surface
%u=-u;
%% SuperTwisitng
smode=abs(s)^alfa;
N4=tanh(s/fi1);
P1=k1*N4*smode;
P2=k2*N44;
G=(l/a1)*(P1+P2);% tanhs replace by sign
u=(-Fr)+(Fext)+100*dote-((Fextc)-(G))*(m);% for sign and tanh
%u=(-Fr)+(Fext)-((Fextc)-(G))*(m);% for sign and tanh
u=-u;
end

% disp(['Input 1: ', num2str(input1_value), ', Input 2: ', num2str(input2_value)]);
% disp(['Output b: ', num2str(output_values(1)), ', Output c: ', num2str(output_values(2))]);

== matlab function ellipsoidSMC/Rigid Body/Hydrodynamic Body/Wave Diffraction and Excitation Force Calculation/Linear Wave Excitation Force Variant Subsystem/Irregular Wave NonLinearYaw/MATLAB Function ==
  data: A input; w input; dofGRD input; dirGRD input; wGRD input; fEHRE input; fEHIM input; Fext output; fEHMD input; phaseRand input; dw input; time input; direction input; spread input; Disp input; intThresh input; prevYaw input; relYawLast output; prevCoeffMD input; prevCoeffRE input; prevCoeffIM input; coeffsLastMD output; coeffsLastRE output; coeffsLastIM output
function [Fext,relYawLast,coeffsLastMD,coeffsLastRE,coeffsLastIM] = irregnLYaw(A,w,dofGRD,dirGRD,wGRD,fEHRE,fEHIM, fEHMD, phaseRand,dw,time,direction,spread, Disp, intThresh, prevYaw, prevCoeffMD, prevCoeffRE, prevCoeffIM)

%initialize outputs
Fext = zeros(1,6);
relYawLast=0;
coeffsLastMD=zeros(length(w),6);
coeffsLastRE=zeros(length(w),6);
coeffsLastIM=zeros(length(w),6);

[Fext,relYawLast,coeffsLastMD,coeffsLastRE,coeffsLastIM] = irregnLYaw(A,w,dofGRD,dirGRD,wGRD,fEHRE,fEHIM, fEHMD, phaseRand,dw,time,direction,spread, Disp, intThresh, prevYaw, prevCoeffMD, prevCoeffRE, prevCoeffIM);

end
